simulink library "cntrlAttiRedIndi_lib"  (R2018b)
settings: Solver=VariableStepAuto  StartTime=0.0  StopTime=10.0  RelTol=1e-3
undefined symbols (not defined in the file or in its folder): atc, DiscIntNeverNeededParam
libraries: angles_lib x3, filters_lib x2, axes_transformation_lib x1, ndi_lib x1
settings Model: Creator=Ybeyer  LastModifiedBy=yannic
settings SFSimCC: SimUseLocalCustomCode=off
settings RTWCC: RTWUseLocalCustomCode=off
settings CodeAppCC: StateflowObjectComments=on

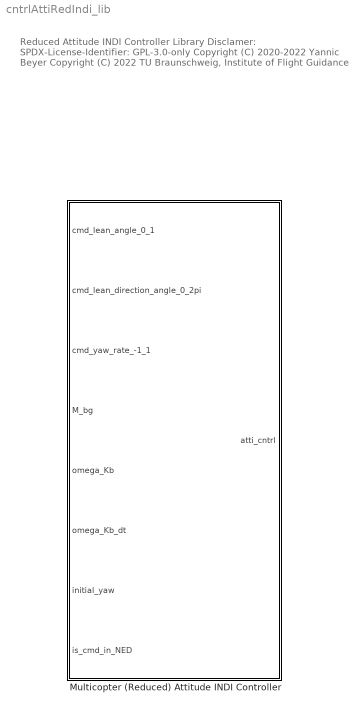
== system cntrlAttiRedIndi_lib ==
  note: Reduced Attitude INDI Controller Library
      |
      | Disclamer:
      | SPDX-License-Identifier: GPL-3.0-only
      |
      | Copyright (C) 2020-2022 Yannic Beyer
      | Copyright (C) 2022 TU Braunschweig, Institute of Flight Guidance
  Multicopter (Reduced) Attitude INDI Controller : Subsystem  mask{atc=atc, T=0.01}
      mask prompts: atc "reduced attitude control parameters struct, see cntrlAttiRedIndi_params_default"; T "inner loop time constant"
      mask Help: https://www.mathworks.com
      mask DialogControl DescGroupVar Prompt: INDI Reduced Attitude Controller

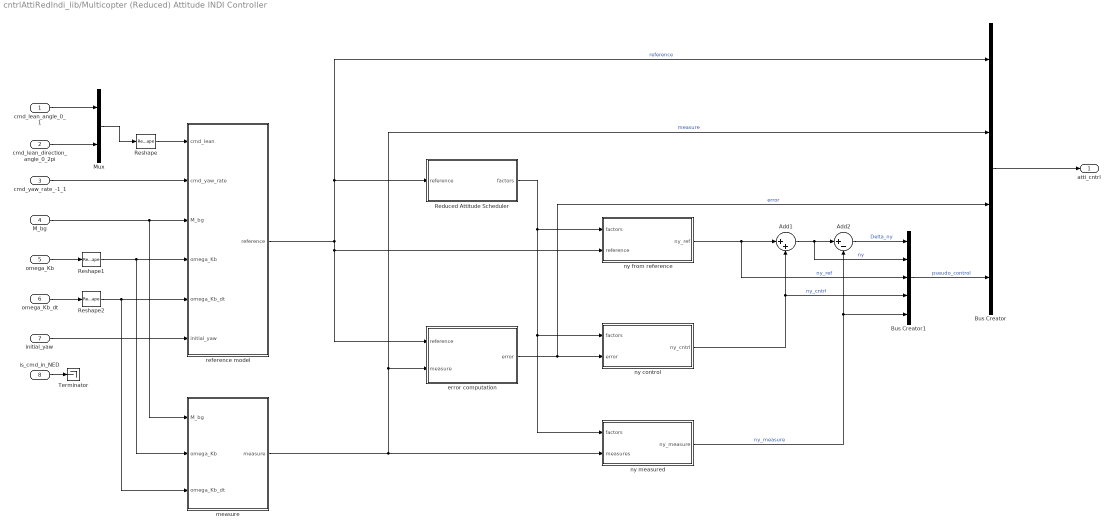
== system cntrlAttiRedIndi_lib/Multicopter (Reduced) Attitude INDI Controller ==
  cmd_lean_angle_0_1 : Inport
  cmd_lean_direction_angle_0_2pi : Inport  Port=2
  cmd_yaw_rate_-1_1 : Inport  Port=3
  M_bg : Inport  Port=4
  omega_Kb : Inport  Port=5
  omega_Kb_dt : Inport  Port=6
  initial_yaw : Inport  Port=7
  is_cmd_in_NED : Inport  Port=8
  Add1 : Sum  Inputs=|++
  Add2 : Sum  Inputs=|+-
  Bus Creator : BusCreator  Inputs=4
  Bus Creator1 : BusCreator  Inputs=5
  Mux : Mux  Inputs=2
  Reduced Attitude Scheduler : Subsystem
  Reshape : Reshape  OutputDimensionality=Column vector (2-D)
  Reshape1 : Reshape  OutputDimensionality=Column vector (2-D)
  Reshape2 : Reshape  OutputDimensionality=Column vector (2-D)
  Terminator : Terminator
  error computation : Subsystem
  measure : Subsystem
  ny control : Subsystem
  ny from reference : Subsystem
  ny measured : Subsystem
  reference model : Subsystem
  atti_cntrl : Outport
  wires:
  ny from reference/1(ny_ref) -> Bus Creator1/3, Add1/1  "ny_ref"
  Mux/1 -> Reshape/1
  error computation/1(error) -> ny control/2(error), Bus Creator/3  "error"
  omega_Kb_dt/1 -> Reshape2/1
  ny control/1(ny_cntrl) -> Add1/2, Bus Creator1/4  "ny_cntrl"
  ny measured/1(ny_measure) -> Bus Creator1/5, Add2/2  "ny_measure"
  reference model/1(reference) -> error computation/1(reference), ny from reference/2(reference), Reduced Attitude Scheduler/1(reference), Bus Creator/1  "reference"
  initial_yaw/1 -> reference model/6(initial_yaw)
  Bus Creator/1 -> atti_cntrl/1
  Bus Creator1/1 -> Bus Creator/4  "pseudo_control"
  Add2/1 -> Bus Creator1/1  "Delta_ny"
  M_bg/1 -> reference model/3(M_bg), measure/1(M_bg)
  omega_Kb/1 -> Reshape1/1
  measure/1(measure) -> Bus Creator/2, error computation/2(measure), ny measured/2(measures)  "measure"
  Reshape/1 -> reference model/1(cmd_lean)
  Reshape1/1 -> reference model/4(omega_Kb), measure/2(omega_Kb)
  Reshape2/1 -> reference model/5(omega_Kb_dt), measure/3(omega_Kb_dt)
  cmd_lean_angle_0_1/1 -> Mux/1
  cmd_lean_direction_angle_0_2pi/1 -> Mux/2
  cmd_yaw_rate_-1_1/1 -> reference model/2(cmd_yaw_rate)
  is_cmd_in_NED/1 -> Terminator/1
  Add1/1 -> Bus Creator1/2, Add2/1  "ny"
  Reduced Attitude Scheduler/1(factors) -> ny measured/1(factors), ny control/1(factors), ny from reference/1(factors)

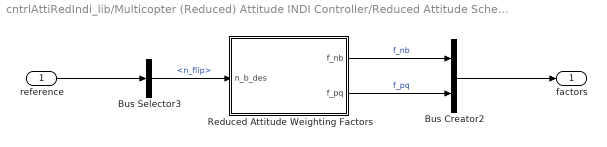
== system cntrlAttiRedIndi_lib/Multicopter (Reduced) Attitude INDI Controller/Reduced Attitude Scheduler ==
  reference : Inport
  Bus Creator2 : BusCreator  Inputs=2
  Bus Selector3 : BusSelector  OutputSignals=reduced_attitude.n_flip
  Reduced Attitude Weighting Factors : MATLAB Function  TreatAsAtomicUnit=on
  factors : Outport
  wires:
  Bus Selector3/1 -> Reduced Attitude Weighting Factors/1(n_b_des)  "<n_flip>"
  Reduced Attitude Weighting Factors/1(f_nb) -> Bus Creator2/1  "f_nb"
  Reduced Attitude Weighting Factors/2(f_pq) -> Bus Creator2/2  "f_pq"
  reference/1 -> Bus Selector3/1
  Bus Creator2/1 -> factors/1

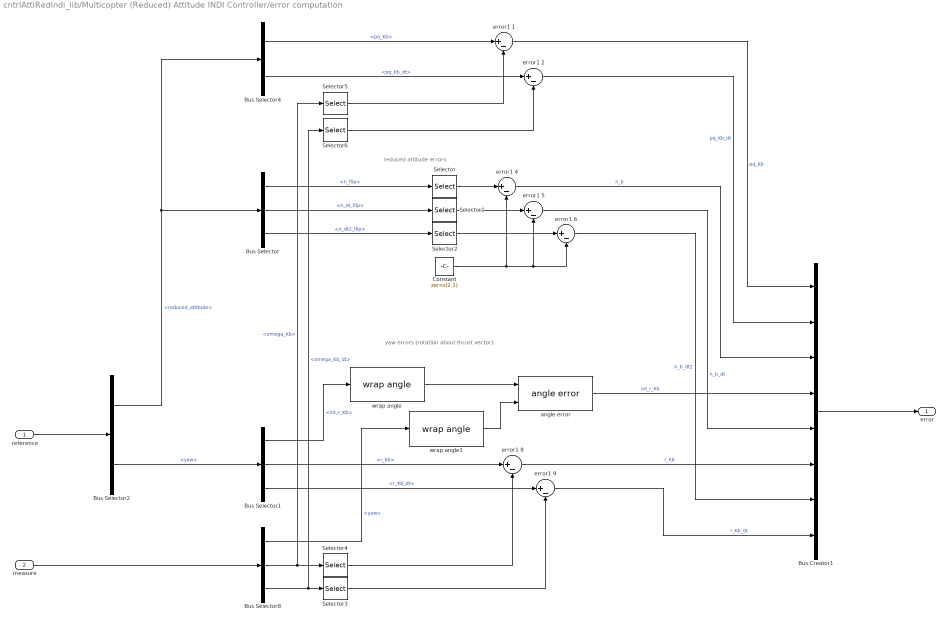
== system cntrlAttiRedIndi_lib/Multicopter (Reduced) Attitude INDI Controller/error computation ==
  note: reduced attitude errors
  note: yaw errors (rotation about thrust vector)
  reference : Inport
  measure : Inport  Port=2
  Bus Creator1 : BusCreator  Inputs=8
  Bus Selector : BusSelector  OutputSignals=n_flip,n_dt_flip,n_dt2_flip
  Bus Selector1 : BusSelector  OutputSignals=int_r_Kb,r_Kb,r_Kb_dt
  Bus Selector2 : BusSelector  OutputSignals=reduced_attitude,yaw
  Bus Selector4 : BusSelector  OutputSignals=pq_Kb,pq_Kb_dt
  Bus Selector8 : BusSelector  OutputSignals=yaw,omega_Kb,omega_Kb_dt
  Constant : Constant  Value=zeros(2,1)
  Selector : Selector  InputPortWidth=3  IndexOptions=Index vector (dialog)  Indices=[1,2]  OutputSizes=1
  Selector1 : Selector  InputPortWidth=3  IndexOptions=Index vector (dialog)  Indices=[1,2]  OutputSizes=1
  Selector2 : Selector  InputPortWidth=3  IndexOptions=Index vector (dialog)  Indices=[1,2]  OutputSizes=1
  Selector3 : Selector  InputPortWidth=3  IndexOptions=Index vector (dialog)  Indices=3  OutputSizes=1
  Selector4 : Selector  InputPortWidth=3  IndexOptions=Index vector (dialog)  Indices=3  OutputSizes=1
  Selector5 : Selector  InputPortWidth=3  IndexOptions=Index vector (dialog)  Indices=1:2  OutputSizes=1
  Selector6 : Selector  InputPortWidth=3  IndexOptions=Index vector (dialog)  Indices=1:2  OutputSizes=1
  angle error : angles_lib/angle error  SystemSampleTime=-1
      settings: SourceProductName=LADAC
  error1 {1..2,4..6,8..9} (7 alike) : Sum  Inputs=|+-
  wrap angle : angles_lib/wrap angle  SystemSampleTime=-1
      settings: SourceProductName=LADAC
  wrap angle1 : angles_lib/wrap angle  SystemSampleTime=-1
      settings: SourceProductName=LADAC
  error : Outport
  wires:
  error1 4/1 -> Bus Creator1/3  "n_b"
  reference/1 -> Bus Selector2/1
  Bus Selector/1 -> Selector/1  "<n_flip>"
  Bus Selector/2 -> Selector1/1  "<n_dt_flip>"
  Bus Selector/3 -> Selector2/1  "<n_dt2_flip>"
  Bus Selector2/1 -> Bus Selector4/1, Bus Selector/1  "<reduced_attitude>"
  Bus Creator1/1 -> error/1
  Selector/1 -> error1 4/1
  Selector1/1 -> error1 5/1
  Selector2/1 -> error1 6/1
  Constant/1 -> error1 6/2, error1 5/2, error1 4/2
  Bus Selector2/2 -> Bus Selector1/1  "<yaw>"
  Bus Selector1/1 -> wrap angle/1  "<int_r_Kb>"
  Bus Selector1/2 -> error1 8/1  "<r_Kb>"
  Bus Selector1/3 -> error1 9/1  "<r_Kb_dt>"
  measure/1 -> Bus Selector8/1
  Bus Selector8/3 -> Selector6/1, Selector3/1  "<omega_Kb_dt>"
  Bus Selector8/2 -> Selector4/1, Selector5/1  "<omega_Kb>"
  Bus Selector8/1 -> wrap angle1/1  "<yaw>"
  Selector4/1 -> error1 8/2
  Selector3/1 -> error1 9/2
  angle error/1 -> Bus Creator1/4  "int_r_Kb"
  error1 8/1 -> Bus Creator1/6  "r_Kb"
  error1 5/1 -> Bus Creator1/5  "n_b_dt"
  error1 6/1 -> Bus Creator1/7  "n_b_dt2"
  error1 9/1 -> Bus Creator1/8  "r_Kb_dt"
  wrap angle1/1 -> angle error/2
  wrap angle/1 -> angle error/1
  Bus Selector4/1 -> error1 1/1  "<pq_Kb>"
  Bus Selector4/2 -> error1 2/1  "<pq_Kb_dt>"
  error1 1/1 -> Bus Creator1/1  "pq_Kb"
  Selector5/1 -> error1 1/2
  Selector6/1 -> error1 2/2
  error1 2/1 -> Bus Creator1/2  "pq_Kb_dt"

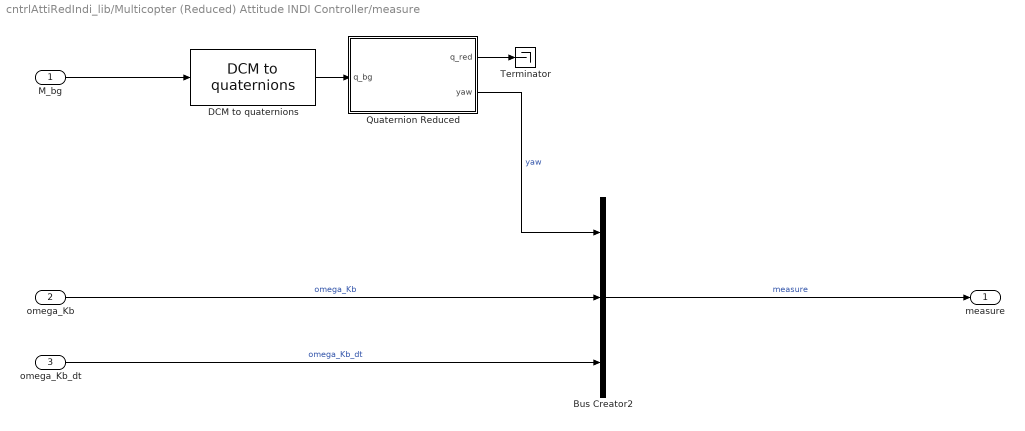
== system cntrlAttiRedIndi_lib/Multicopter (Reduced) Attitude INDI Controller/measure ==
  M_bg : Inport
  omega_Kb : Inport  Port=2
  omega_Kb_dt : Inport  Port=3
  Bus Creator2 : BusCreator  Inputs=3
  DCM to quaternions : axes_transformation_lib/DCM to quaternions  SystemSampleTime=-1
      settings: SourceProductName=LADAC
  Quaternion Reduced : MATLAB Function  TreatAsAtomicUnit=on
  Terminator : Terminator
  measure : Outport
  wires:
  DCM to quaternions/1 -> Quaternion Reduced/1(q_bg)
  Quaternion Reduced/1(q_red) -> Terminator/1
  Quaternion Reduced/2(yaw) -> Bus Creator2/1  "yaw"
  M_bg/1 -> DCM to quaternions/1
  omega_Kb/1 -> Bus Creator2/2  "omega_Kb"
  omega_Kb_dt/1 -> Bus Creator2/3  "omega_Kb_dt"
  Bus Creator2/1 -> measure/1  "measure"

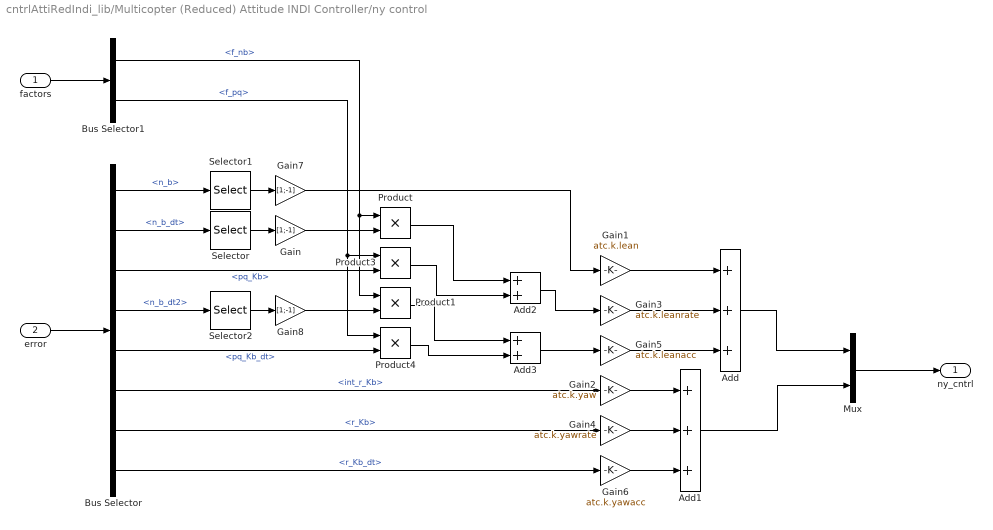
== system cntrlAttiRedIndi_lib/Multicopter (Reduced) Attitude INDI Controller/ny control ==
  factors : Inport
  error : Inport  Port=2
  Add : Sum  Inputs=3
  Add1 : Sum  Inputs=3
  Add2 : Sum
  Add3 : Sum
  Bus Selector : BusSelector  OutputSignals=n_b,n_b_dt,pq_Kb,n_b_dt2,pq_Kb_dt,int_r_Kb,r_Kb,r_Kb_dt
  Bus Selector1 : BusSelector  OutputSignals=f_nb,f_pq
  Gain : Gain  Gain=[1;-1]
  Gain1 : Gain  Gain=atc.k.lean
  Gain2 : Gain  Gain=atc.k.yaw
  Gain3 : Gain  Gain=atc.k.leanrate
  Gain4 : Gain  Gain=atc.k.yawrate
  Gain5 : Gain  Gain=atc.k.leanacc
  Gain6 : Gain  Gain=atc.k.yawacc
  Gain7 : Gain  Gain=[1;-1]
  Gain8 : Gain  Gain=[1;-1]
  Mux : Mux  Inputs=2
  Product{,1,3..4} (4 alike) : Product
  Selector : Selector  InputPortWidth=2  IndexOptions=Index vector (dialog)  Indices=[2,1]  OutputSizes=1
  Selector1 : Selector  InputPortWidth=2  IndexOptions=Index vector (dialog)  Indices=[2,1]  OutputSizes=1
  Selector2 : Selector  InputPortWidth=2  IndexOptions=Index vector (dialog)  Indices=[2,1]  OutputSizes=1
  ny_cntrl : Outport
  wires:
  error/1 -> Bus Selector/1
  Bus Selector/1 -> Selector1/1  "<n_b>"
  Bus Selector/6 -> Gain2/1  "<int_r_Kb>"
  Bus Selector/2 -> Selector/1  "<n_b_dt>"
  Bus Selector/7 -> Gain4/1  "<r_Kb>"
  Bus Selector/4 -> Selector2/1  "<n_b_dt2>"
  Bus Selector/8 -> Gain6/1  "<r_Kb_dt>"
  Gain5/1 -> Add/3
  Gain3/1 -> Add/2
  Gain1/1 -> Add/1
  Gain2/1 -> Add1/1
  Gain4/1 -> Add1/2
  Gain6/1 -> Add1/3
  Mux/1 -> ny_cntrl/1
  Add1/1 -> Mux/2
  Add/1 -> Mux/1
  Selector/1 -> Gain/1
  factors/1 -> Bus Selector1/1
  Bus Selector1/1 -> Product1/1, Product/1  "<f_nb>"
  Add2/1 -> Gain3/1
  Bus Selector/3 -> Product3/2  "<pq_Kb>"
  Add3/1 -> Gain5/1
  Product/1 -> Add2/1
  Product1/1 -> Add3/1
  Bus Selector1/2 -> Product4/1, Product3/1  "<f_pq>"
  Bus Selector/5 -> Product4/2  "<pq_Kb_dt>"
  Product4/1 -> Add3/2
  Product3/1 -> Add2/2
  Gain/1 -> Product/2
  Selector1/1 -> Gain7/1
  Gain7/1 -> Gain1/1
  Selector2/1 -> Gain8/1
  Gain8/1 -> Product1/2

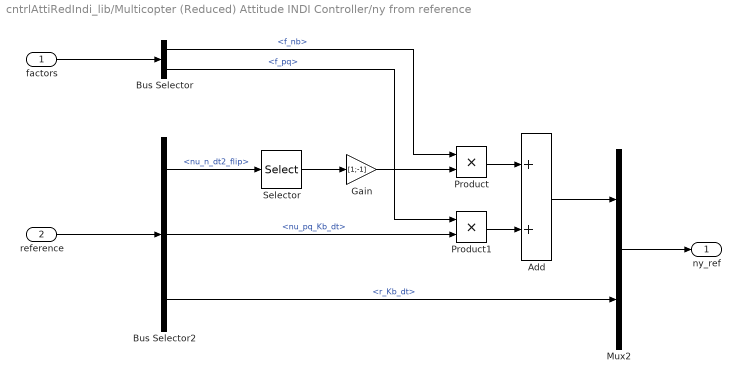
== system cntrlAttiRedIndi_lib/Multicopter (Reduced) Attitude INDI Controller/ny from reference ==
  factors : Inport
  reference : Inport  Port=2
  Add : Sum
  Bus Selector : BusSelector  OutputSignals=f_nb,f_pq
  Bus Selector2 : BusSelector  OutputSignals=reduced_attitude.nu_n_dt2_flip,reduced_attitude.nu_pq_Kb_dt,yaw.r_Kb_dt
  Gain : Gain  Gain=[1;-1]
  Mux2 : Mux  Inputs=2
  Product : Product
  Product1 : Product
  Selector : Selector  InputPortWidth=3  IndexOptions=Index vector (dialog)  Indices=[2,1]  OutputSizes=1
  ny_ref : Outport
  wires:
  Mux2/1 -> ny_ref/1
  Bus Selector2/3 -> Mux2/2  "<r_Kb_dt>"
  Bus Selector2/1 -> Selector/1  "<nu_n_dt2_flip>"
  Selector/1 -> Gain/1
  Gain/1 -> Product/2
  reference/1 -> Bus Selector2/1
  Bus Selector/1 -> Product/1  "<f_nb>"
  Product/1 -> Add/1
  Bus Selector2/2 -> Product1/2  "<nu_pq_Kb_dt>"
  Bus Selector/2 -> Product1/1  "<f_pq>"
  Product1/1 -> Add/2
  Add/1 -> Mux2/1
  factors/1 -> Bus Selector/1

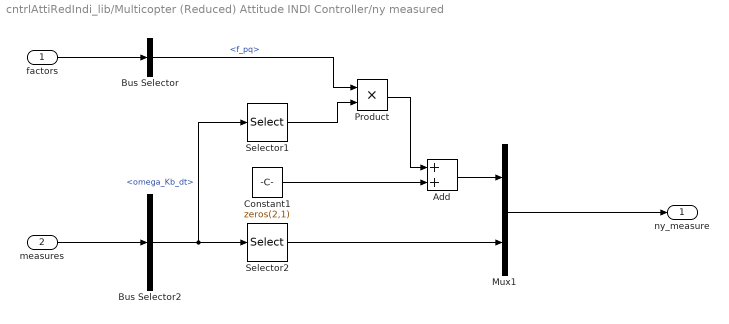
== system cntrlAttiRedIndi_lib/Multicopter (Reduced) Attitude INDI Controller/ny measured ==
  factors : Inport
  measures : Inport  Port=2
  Add : Sum
  Bus Selector : BusSelector  OutputSignals=f_pq
  Bus Selector2 : BusSelector  OutputSignals=omega_Kb_dt
  Constant1 : Constant  Value=zeros(2,1)
  Mux1 : Mux  Inputs=2
  Product : Product
  Selector1 : Selector  InputPortWidth=3  IndexOptions=Index vector (dialog)  Indices=1:2  OutputSizes=1
  Selector2 : Selector  InputPortWidth=3  IndexOptions=Index vector (dialog)  Indices=3  OutputSizes=1
  ny_measure : Outport
  wires:
  Bus Selector2/1 -> Selector2/1, Selector1/1  "<omega_Kb_dt>"
  measures/1 -> Bus Selector2/1
  Mux1/1 -> ny_measure/1
  Selector2/1 -> Mux1/2
  Constant1/1 -> Add/2
  factors/1 -> Bus Selector/1
  Bus Selector/1 -> Product/1  "<f_pq>"
  Selector1/1 -> Product/2
  Add/1 -> Mux1/1
  Product/1 -> Add/1

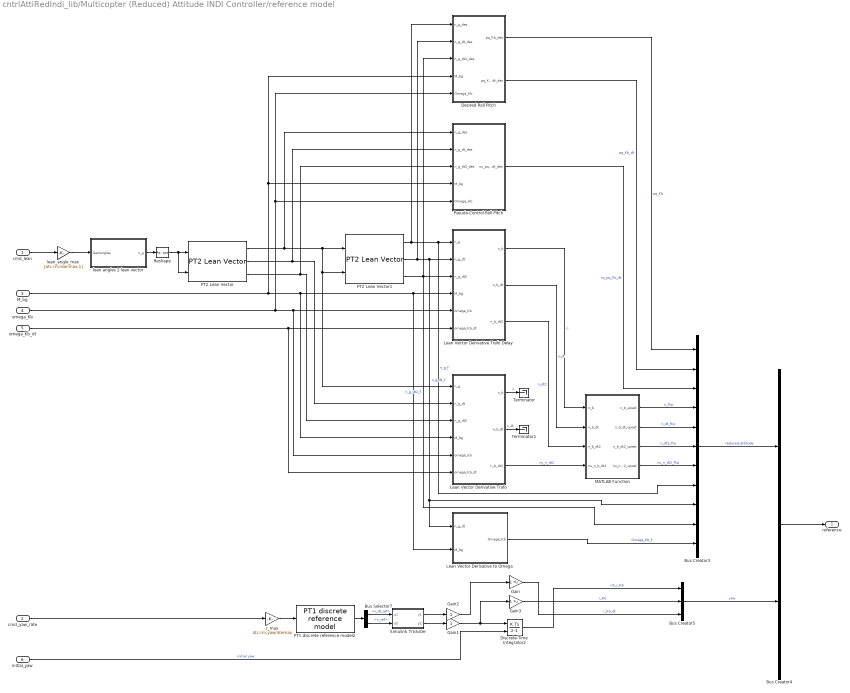
== system cntrlAttiRedIndi_lib/Multicopter (Reduced) Attitude INDI Controller/reference model ==
  cmd_lean : Inport
  cmd_yaw_rate : Inport  Port=2
  M_bg : Inport  Port=3
  omega_Kb : Inport  Port=4
  omega_Kb_dt : Inport  Port=5
  initial_yaw : Inport  Port=6
  Bus Creator3 : BusCreator  Inputs=11
  Bus Creator4 : BusCreator  Inputs=2
  Bus Creator5 : BusCreator  Inputs=3
  Bus Selector7 : BusSelector  OutputSignals=x_dt_ref,x_ref
  Desired Roll Pitch : MATLAB Function  TreatAsAtomicUnit=on
  Discrete-Time Integrator2 : DiscreteIntegrator  InitialConditionSource=external  SampleTime=-1  ICPrevOutput=DiscIntNeverNeededParam  ICPrevScaledInput=DiscIntNeverNeededParam
  Gain : Gain  Multiplication=Matrix(K*u)
  Gain1 : Gain
  Gain2 : Gain
  Gain3 : Gain  Multiplication=Matrix(K*u)
  Lean Vector Derivative Trafo : MATLAB Function  TreatAsAtomicUnit=on
  Lean Vector Derivative Trafo Delay : MATLAB Function  TreatAsAtomicUnit=on
  Lean Vector Derivative to Omega : MATLAB Function  TreatAsAtomicUnit=on
  MATLAB Function : MATLAB Function  TreatAsAtomicUnit=on
  PT1 discrete reference model2 : ndi_lib/PT1 discrete reference model  T=atc.rm.yawratetc  x_max=inf  x_min=-inf  x_dt_max=inf  x_dt_min=-inf  x_init=0
      settings: SourceProductName=LADAC
  PT2 Lean Vector : filters_lib/PT2 Lean Vector  omega=atc.rm.leanfreq  d=atc.rm.leandamp  x_dt2_max=inf  x_dt2_min=-inf  x_dt_max=inf  x_dt_min=-inf  x_max=inf  x_min=-inf  x_init=0  x_dt_init=0
      settings: SourceProductName=LADAC
  PT2 Lean Vector1 : filters_lib/PT2 Lean Vector  omega=2./T  d=1  x_dt2_max=inf  x_dt2_min=-inf  x_dt_max=inf  x_dt_min=-inf  x_max=inf  x_min=-inf  x_init=0  x_dt_init=0
      settings: SourceProductName=LADAC
  Pseudo-Control Roll Pitch : MATLAB Function  TreatAsAtomicUnit=on
  Reshape : Reshape  OutputDimensionality=Column vector (2-D)
  Simulink Trickster : MATLAB Function  TreatAsAtomicUnit=on
  Terminator : Terminator
  Terminator1 : Terminator
  lean angles 2 lean vector : MATLAB Function  TreatAsAtomicUnit=on
  lean_angle_max : Gain  Gain=[atc.rm.leanmax;1]
  r_max : Gain  Gain=atc.rm.yawratemax
  reference : Outport
  wires:
  initial_yaw/1 -> Discrete-Time Integrator2/2  "initial yaw"
  Lean Vector Derivative Trafo/3(n_b_dt2) -> MATLAB Function/4(nu_n_b_dt2)  "ny_n_dt2"
  Lean Vector Derivative Trafo Delay/2(n_b_dt) -> MATLAB Function/2(n_b_dt)  "n_dt"
  Lean Vector Derivative Trafo Delay/1(n_b) -> MATLAB Function/1(n_b)  "n"
  lean angles 2 lean vector/1(n_g) -> Reshape/1
  Bus Creator4/1 -> reference/1
  Bus Creator3/1 -> Bus Creator4/1  "reduced_attitude"
  cmd_yaw_rate/1 -> r_max/1
  r_max/1 -> PT1 discrete reference model2/1
  PT1 discrete reference model2/1 -> Bus Selector7/1
  Bus Creator5/1 -> Bus Creator4/2  "yaw"
  Discrete-Time Integrator2/1 -> Bus Creator5/1  "int_r_Kb"
  Gain/1 -> Bus Creator5/3  "r_Kb_dt"
  Gain3/1 -> Bus Creator5/2  "r_Kb"
  lean_angle_max/1 -> lean angles 2 lean vector/1(leanAngles)
  Lean Vector Derivative Trafo Delay/3(n_b_dt2) -> MATLAB Function/3(n_b_dt2)  "n_dt2"
  Lean Vector Derivative Trafo/1(n_b) -> Terminator/1  "n"
  Lean Vector Derivative Trafo/2(n_b_dt) -> Terminator1/1  "n_dt"
  PT2 Lean Vector/1 -> PT2 Lean Vector1/1, PT2 Lean Vector1/2, Lean Vector Derivative Trafo/1(n_g), Pseudo-Control Roll Pitch/1(n_g_des)
  PT2 Lean Vector1/1 -> Lean Vector Derivative Trafo Delay/1(n_g), Bus Creator3/8, Desired Roll Pitch/1(n_g_des)  "n_g_f"
  PT2 Lean Vector1/2 -> Lean Vector Derivative Trafo Delay/2(n_g_dt), Lean Vector Derivative to Omega/1(n_g_dt), Bus Creator3/9, Desired Roll Pitch/2(n_g_dt_des)  "n_g_dt_f"
  PT2 Lean Vector1/3 -> Bus Creator3/10, Desired Roll Pitch/3(n_g_dt2_des), Lean Vector Derivative Trafo Delay/3(n_g_dt2)  "n_g_dt2_f"
  MATLAB Function/1(n_b_upset) -> Bus Creator3/4  "n_flip"
  MATLAB Function/2(n_b_dt_upset) -> Bus Creator3/5  "n_dt_flip"
  MATLAB Function/3(n_b_dt2_upset) -> Bus Creator3/6  "n_dt2_flip"
  MATLAB Function/4(nu_n_b_dt2_upset) -> Bus Creator3/7  "nu_n_dt2_flip"
  omega_Kb_dt/1 -> Lean Vector Derivative Trafo Delay/6(omega_Kb_dt), Lean Vector Derivative Trafo/6(omega_Kb_dt)
  omega_Kb/1 -> Lean Vector Derivative Trafo/5(omega_Kb), Lean Vector Derivative Trafo Delay/5(omega_Kb), Pseudo-Control Roll Pitch/5(Omega_Kb), Desired Roll Pitch/5(Omega_Kb)
  M_bg/1 -> Lean Vector Derivative Trafo Delay/4(M_bg), Lean Vector Derivative to Omega/2(M_bg), Lean Vector Derivative Trafo/4(M_bg), Desired Roll Pitch/4(M_bg), Pseudo-Control Roll Pitch/4(M_bg)
  PT2 Lean Vector/3 -> Pseudo-Control Roll Pitch/3(n_g_dt2_des), Lean Vector Derivative Trafo/3(n_g_dt2)
  PT2 Lean Vector/2 -> Pseudo-Control Roll Pitch/2(n_g_dt_des), Lean Vector Derivative Trafo/2(n_g_dt)
  Reshape/1 -> PT2 Lean Vector/2, PT2 Lean Vector/1
  cmd_lean/1 -> lean_angle_max/1
  Lean Vector Derivative to Omega/1(Omega_Kb) -> Bus Creator3/11  "Omega_Kb_f"
  Gain1/1 -> Gain3/1, Discrete-Time Integrator2/1
  Gain2/1 -> Gain/1
  Simulink Trickster/1(y1) -> Gain2/1
  Simulink Trickster/2(y2) -> Gain1/1
  Bus Selector7/1 -> Simulink Trickster/1(u1)  "<x_dt_ref>"
  Bus Selector7/2 -> Simulink Trickster/2(u2)  "<x_ref>"
  Desired Roll Pitch/2(pq_Kb_dt_des) -> Bus Creator3/2  "pq_Kb_dt"
  Desired Roll Pitch/1(pq_Kb_des) -> Bus Creator3/1  "pq_Kb"
  Pseudo-Control Roll Pitch/1(nu_pq_Kb_dt_des) -> Bus Creator3/3  "nu_pq_Kb_dt"

== matlab function cntrlAttiRedIndi_lib/Multicopter (Reduced) Attitude INDI Controller/reference model/Lean Vector Derivative Trafo Delay ==
  data: n_g input; n_b output; n_g_dt input; n_g_dt2 input; M_bg input; omega_Kb input; omega_Kb_dt input; n_b_dt output; n_b_dt2 output
function [ n_b, n_b_dt, n_b_dt2 ] = leanVectorDerivTrafo( n_g, n_g_dt, ...
    n_g_dt2, M_bg, omega_Kb, omega_Kb_dt )
[ n_b, n_b_dt, n_b_dt2 ] = leanVectorDerivTrafo( n_g, n_g_dt, ...
    n_g_dt2, M_bg, omega_Kb, omega_Kb_dt );
end

== matlab function cntrlAttiRedIndi_lib/Multicopter (Reduced) Attitude INDI Controller/reference model/MATLAB Function ==
  data: n_b input; n_b_upset output; n_b_dt input; n_b_dt2 input; n_b_dt_upset output; n_b_dt2_upset output; nu_n_b_dt2 input; nu_n_b_dt2_upset output
function [ n_b_upset, n_b_dt_upset, n_b_dt2_upset, nu_n_b_dt2_upset ] = ...
    indiCopterLeanVectorUpset( n_b, n_b_dt, n_b_dt2, nu_n_b_dt2 )
[ n_b_upset, n_b_dt_upset, n_b_dt2_upset, nu_n_b_dt2_upset ] = ...
    indiCopterLeanVectorUpset( n_b, n_b_dt, n_b_dt2, nu_n_b_dt2 );
end

== matlab function cntrlAttiRedIndi_lib/Multicopter (Reduced) Attitude INDI Controller/reference model/lean angles 2 lean vector ==
  data: leanAngles input; n_g output
function n_g = leanAngles2leanVector( leanAngles )
n_g = leanAngles2leanVector( leanAngles );
end

== matlab function cntrlAttiRedIndi_lib/Multicopter (Reduced) Attitude INDI Controller/reference model/Lean Vector Derivative Trafo ==
  data: n_g input; n_b output; n_g_dt input; n_g_dt2 input; M_bg input; omega_Kb input; omega_Kb_dt input; n_b_dt output; n_b_dt2 output
function [ n_b, n_b_dt, n_b_dt2 ] = leanVectorDerivTrafo( n_g, n_g_dt, ...
    n_g_dt2, M_bg, omega_Kb, omega_Kb_dt )
[ n_b, n_b_dt, n_b_dt2 ] = leanVectorDerivTrafo( n_g, n_g_dt, ...
    n_g_dt2, M_bg, omega_Kb, omega_Kb_dt );
end

== matlab function cntrlAttiRedIndi_lib/Multicopter (Reduced) Attitude INDI Controller/reference model/Simulink Trickster ==
  data: u1 input size=1; y1 output size=1; u2 input size=1; y2 output size=1
function [y1,y2] = fcn(u1,u2)
% I cried a lot and prayed often to the Simulink god.
% But this was the best solution I could find for a Simulink dimensions error.
% Note that the dimensions of u1, u2, y1, y2 are hard coded in the Model
% Explorer.
y1 = u1;
y2 = u2;
end

== matlab function cntrlAttiRedIndi_lib/Multicopter (Reduced) Attitude INDI Controller/reference model/Pseudo-Control Roll Pitch ==
  data: n_g_des input; n_g_dt_des input; n_g_dt2_des input; nu_pq_Kb_dt_des output; M_bg input; Omega_Kb input
function nu_pq_Kb_dt_des  = fcn(n_g_des,n_g_dt_des,n_g_dt2_des,M_bg,Omega_Kb)
Omega_Kg_des = cross(n_g_des,n_g_dt_des);
Omega_Kg_dt_des = cross(n_g_des,n_g_dt2_des);
M_bg_dt = dcmDerivFromOmega(M_bg',Omega_Kb)';
Omega_Kb_dt_des = M_bg * Omega_Kg_dt_des + M_bg_dt * Omega_Kg_des;
nu_pq_Kb_dt_des = Omega_Kb_dt_des(1:2);
end

== matlab function cntrlAttiRedIndi_lib/Multicopter (Reduced) Attitude INDI Controller/Reduced Attitude Scheduler/Reduced Attitude Weighting Factors ==
  data: f_nb output; n_b_des input; f_pq output
function [f_nb,f_pq] = fcn(n_b_des)

n_b_perfect = n_b_des;
n_b_perfect(:) = [0;0;-1];
f_nb = dot(n_b_des,n_b_perfect);
if f_nb < 0
    f_nb(:) = 0;
end
f_pq = 1 - f_nb;

end

== matlab function cntrlAttiRedIndi_lib/Multicopter (Reduced) Attitude INDI Controller/reference model/Lean Vector Derivative to Omega ==
  data: n_g_dt input; Omega_Kb output; M_bg input
function Omega_Kb = leanVectorDeriv2Omega( n_g_dt, M_bg )
Omega_Kb = leanVectorDeriv2Omega( n_g_dt, M_bg );
end

== matlab function cntrlAttiRedIndi_lib/Multicopter (Reduced) Attitude INDI Controller/measure/Quaternion Reduced ==
  data: q_bg input; q_red output; yaw output
function [q_red,yaw] = fcn(q_bg)
[q_red,yaw] = quatReduced(q_bg);
end

== matlab function cntrlAttiRedIndi_lib/Multicopter (Reduced) Attitude INDI Controller/reference model/Desired Roll Pitch ==
  data: n_g_des input; n_g_dt_des input; n_g_dt2_des input; pq_Kb_des output; M_bg input; pq_Kb_dt_des output; Omega_Kb input
function [pq_Kb_des,pq_Kb_dt_des] = fcn(n_g_des,n_g_dt_des,n_g_dt2_des,M_bg,Omega_Kb)
Omega_Kg_des = cross(n_g_des,n_g_dt_des);
Omega_Kg_dt_des = cross(n_g_des,n_g_dt2_des);
Omega_Kb_des = M_bg * Omega_Kg_des;
M_bg_dt = dcmDerivFromOmega(M_bg',Omega_Kb)';
Omega_Kb_dt_des = M_bg * Omega_Kg_dt_des + M_bg_dt * Omega_Kg_des;
pq_Kb_des = Omega_Kb_des(1:2);
pq_Kb_dt_des = Omega_Kb_dt_des(1:2);
end
